simulink model "untitled"  (R2023b)
settings: Solver=VariableStepAuto  StartTime=0.0  StopTime=10.0  RelTol=1e-3
settings Model: Creator=Liu  LastModifiedBy=Liu

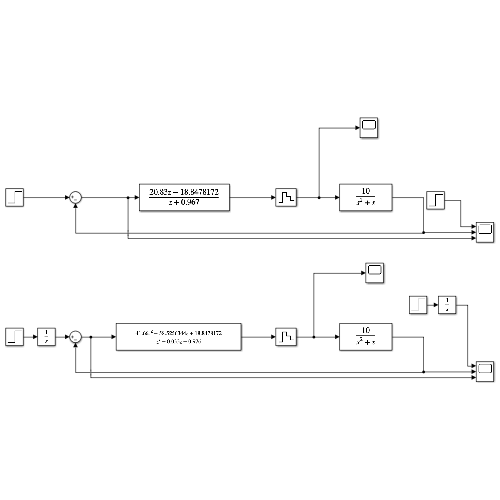
[thumbnail: Simulink's stored preview of the top-level diagram]
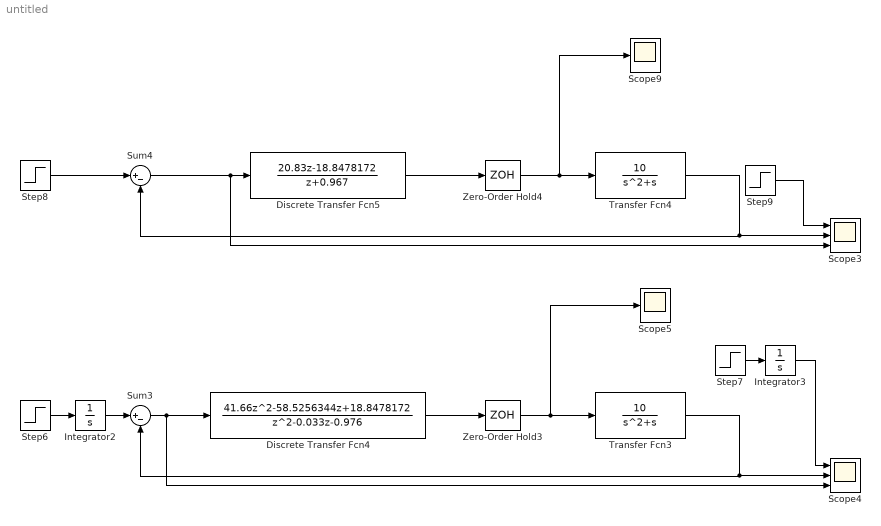
== system untitled ==
  Discrete Transfer Fcn4 : DiscreteTransferFcn  Numerator=[41.66 -58.5256344 18.8478172]  Denominator=[1 -0.033 -0.976]
  Discrete Transfer Fcn5 : DiscreteTransferFcn  Numerator=[20.83 -18.8478172]  Denominator=[1 0.967]
  Integrator2 : Integrator
  Integrator3 : Integrator
  Scope3 : Scope  NumInputPorts=3
  Scope4 : Scope  NumInputPorts=3
  Scope5 : Scope
  Scope9 : Scope
  Step{6..9} (4 alike) : Step  SampleTime=0
  Sum3 : Sum  Inputs=|+-
  Sum4 : Sum  Inputs=|+-
  Transfer Fcn3 : TransferFcn  Numerator=[0 10]  Denominator=[1 1 0]
  Transfer Fcn4 : TransferFcn  Numerator=[0 10]  Denominator=[1 1 0]
  Zero-Order Hold3 : ZeroOrderHold  SampleTime=0.1
  Zero-Order Hold4 : ZeroOrderHold  SampleTime=0.1
  wires:
  Integrator3/1 -> Scope4/1
  Step7/1 -> Integrator3/1
  Step6/1 -> Integrator2/1
  Zero-Order Hold3/1 -> Scope5/1, Transfer Fcn3/1
  Transfer Fcn3/1 -> Sum3/2, Scope4/2
  Sum3/1 -> Discrete Transfer Fcn4/1, Scope4/3
  Discrete Transfer Fcn4/1 -> Zero-Order Hold3/1
  Integrator2/1 -> Sum3/1
  Step8/1 -> Sum4/1
  Step9/1 -> Scope3/1
  Sum4/1 -> Discrete Transfer Fcn5/1, Scope3/3
  Zero-Order Hold4/1 -> Scope9/1, Transfer Fcn4/1
  Discrete Transfer Fcn5/1 -> Zero-Order Hold4/1
  Transfer Fcn4/1 -> Sum4/2, Scope3/2
